simulink model "SIMULINK"  (R2024b)
settings: Solver=FixedStepDiscrete  StartTime=0.0  StopTime=inf  FixedStep=0.01  RelTol=1e-3
undefined symbols (not defined in the file or in its folder): canChannel
libraries: canlib x7, canmsglib x6
settings Model: Creator=sg128629  LastModifiedBy=sg128629

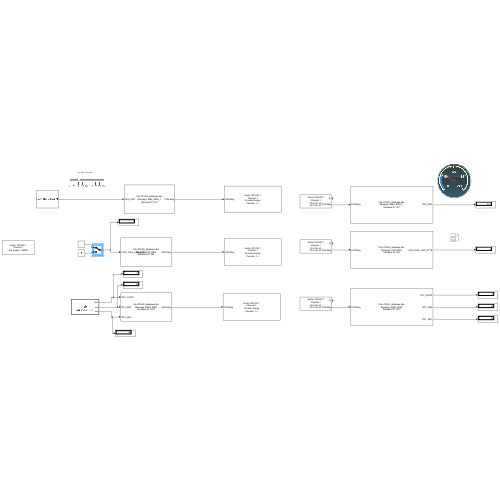
[thumbnail: Simulink's stored preview of the top-level diagram]
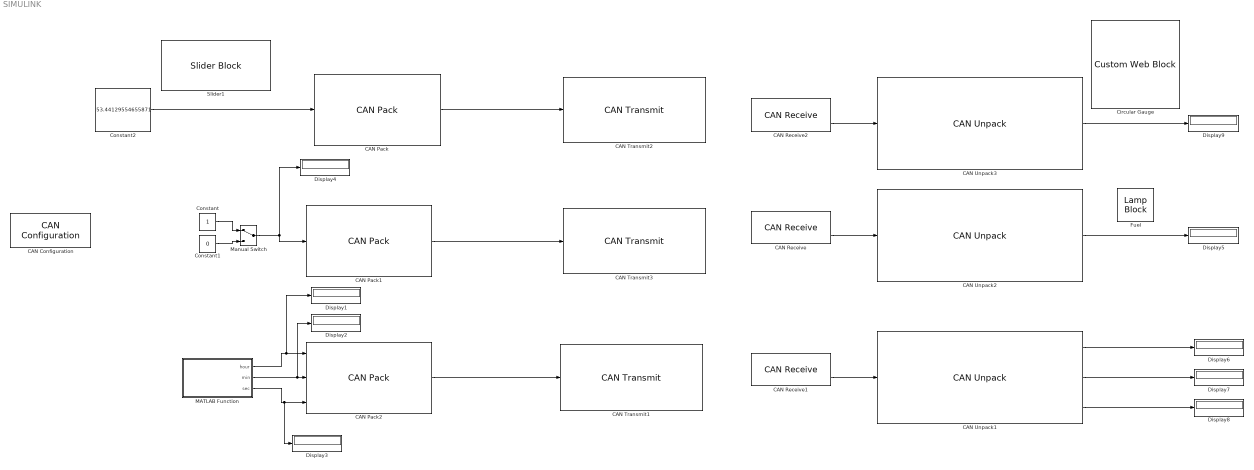
== system SIMULINK ==
  CAN Configuration : canlib/CAN Configuration  BlockHandle=154.0001  Device=Vector VN1630 1 (Channel 1)  DeviceMenu=Vector VN1630 1 (Channel 1)  ObjConstructor=canChannel('Vector', 'VN1630 1', 1)  BusSpeed=125000  EnableBitParameters=off  SJW=1  TSEG1=4  TSEG2=3  NSamples=1  AckMode=Normal
  CAN Pack : canmsglib/CAN Pack  CANdbFile=ATLAS_database.dbc  MsgList=EMS_MSG_1  MsgName=EMS_MSG_1  MsgIDType=Standard (11-bit identifier)  MsgIdentifier=257  CANIDInput=off  MsgLength=8  Remote=off  ApplyMinMax=off  BusOutput=off  SignalInfo={'VEH_SPD','0','12','LE','signed','Standard','0','0.125','0','0','511.625'}
      settings: LibrarySourceBlock=canlib/CAN Pack  DataFormat=CANdb specified signals
  CAN Pack1 : canmsglib/CAN Pack  CANdbFile=ATLAS_database.dbc  MsgList=ICM_MSG  MsgName=ICM_MSG  MsgIDType=Standard (11-bit identifier)  MsgIdentifier=544  CANIDInput=off  MsgLength=8  Remote=off  ApplyMinMax=off  BusOutput=off  SignalInfo={'LOW_FUEL_LMP_STTS','6','2','LE','unsigned','Standard','0','1','0','-Inf','Inf'}
      settings: LibrarySourceBlock=canlib/CAN Pack  DataFormat=CANdb specified signals
  CAN Pack2 : canmsglib/CAN Pack  CANdbFile=ATLAS_database.dbc  MsgList=MMU_MSG  MsgName=MMU_MSG  MsgIDType=Standard (11-bit identifier)  MsgIdentifier=1072  CANIDInput=off  MsgLength=8  Remote=off  ApplyMinMax=off  BusOutput=off  SignalInfo={'RTC_HOUR','16','6','LE','signed','Standard','0','1','0','-Inf','Inf';'RTC_MIN','8','8','LE','signed','Standard','0','1','0','-Inf','Inf';'RTC_SEC','0','8','LE','signed','Standard','0','1','0','-Inf','Inf'}
      settings: LibrarySourceBlock=canlib/CAN Pack  DataFormat=CANdb specified signals
  CAN Receive : canlib/CAN Receive  BlockHandle=166.0001  Device=Vector VN1630 1 (Channel 1)  DeviceMenu=Vector VN1630 1 (Channel 1)  ObjConstructor=canChannel('Vector', 'VN1630 1', 1)  EnableStandardIDsFilter=off  StdIDsCombo=Allow all  StandardIDs=0  EnableExtendedIDsFilter=off  ExtIDsCombo=Allow all  ExtendedIDs=0  SampleTime=0.01  MsgsPerTimestep=1  InternalFilterUpdateStatus=on  BusOutput=off
  CAN Receive1 : canlib/CAN Receive  BlockHandle=169.0001  Device=Vector VN1630 1 (Channel 1)  DeviceMenu=Vector VN1630 1 (Channel 1)  ObjConstructor=canChannel('Vector', 'VN1630 1', 1)  EnableStandardIDsFilter=off  StdIDsCombo=Allow all  StandardIDs=0  EnableExtendedIDsFilter=off  ExtIDsCombo=Allow all  ExtendedIDs=0  SampleTime=0.01  MsgsPerTimestep=1  InternalFilterUpdateStatus=on  BusOutput=off
  CAN Receive2 : canlib/CAN Receive  BlockHandle=172.0001  Device=Vector VN1630 1 (Channel 1)  DeviceMenu=Vector VN1630 1 (Channel 1)  ObjConstructor=canChannel('Vector', 'VN1630 1', 1)  EnableStandardIDsFilter=off  StdIDsCombo=Allow all  StandardIDs=0  EnableExtendedIDsFilter=off  ExtIDsCombo=Allow all  ExtendedIDs=0  SampleTime=0.01  MsgsPerTimestep=1  InternalFilterUpdateStatus=on  BusOutput=off
  CAN Transmit1 : canlib/CAN Transmit  BlockHandle=175.0001  Device=Vector VN1630 1 (Channel 1)  DeviceMenu=Vector VN1630 1 (Channel 1)  ObjConstructor=canChannel('Vector', 'VN1630 1', 1)  EnableEventTransmit=on  EnablePeriodicTransmit=on  MessagePeriod=1.000
  CAN Transmit2 : canlib/CAN Transmit  BlockHandle=177.0001  Device=Vector VN1630 1 (Channel 1)  DeviceMenu=Vector VN1630 1 (Channel 1)  ObjConstructor=canChannel('Vector', 'VN1630 1', 1)  EnableEventTransmit=on  EnablePeriodicTransmit=on  MessagePeriod=1.000
  CAN Transmit3 : canlib/CAN Transmit  BlockHandle=179.0001  Device=Vector VN1630 1 (Channel 1)  DeviceMenu=Vector VN1630 1 (Channel 1)  ObjConstructor=canChannel('Vector', 'VN1630 1', 1)  EnableEventTransmit=on  EnablePeriodicTransmit=on  MessagePeriod=1.000
  CAN Unpack1 : canmsglib/CAN Unpack  CANdbFile=ATLAS_database.dbc  MsgList=MMU_MSG  MsgName=MMU_MSG  MsgIDType=Standard (11-bit identifier)  MsgIdentifier=1072  MsgLength=8  SignalInfo={'RTC_HOUR','16','6','LE','signed','Standard','0','1','0','-Inf','Inf';'RTC_MIN','8','8','LE','signed','Standard','0','1','0','-Inf','Inf';'RTC_SEC','0','8','LE','signed','Standard','0','1','0','-Inf','Inf'}  IDPort=off  TimestampPort=off  ErrorPort=off  RemotePort=off  LengthPort=off  StatusPort=off  ApplyMinMax=off
      settings: LibrarySourceBlock=c2000lib/Target Communication/CAN Unpack  DataFormat=CANdb specified signals
  CAN Unpack2 : canmsglib/CAN Unpack  CANdbFile=ATLAS_database.dbc  MsgList=ICM_MSG  MsgName=ICM_MSG  MsgIDType=Standard (11-bit identifier)  MsgIdentifier=544  MsgLength=8  SignalInfo={'LOW_FUEL_LMP_STTS','6','2','LE','unsigned','Standard','0','1','0','-Inf','Inf'}  IDPort=off  TimestampPort=off  ErrorPort=off  RemotePort=off  LengthPort=off  StatusPort=off  ApplyMinMax=off
      settings: LibrarySourceBlock=c2000lib/Target Communication/CAN Unpack  DataFormat=CANdb specified signals
  CAN Unpack3 : canmsglib/CAN Unpack  CANdbFile=ATLAS_database.dbc  MsgList=EMS_MSG_1  MsgName=EMS_MSG_1  MsgIDType=Standard (11-bit identifier)  MsgIdentifier=257  MsgLength=8  SignalInfo={'VEH_SPD','0','12','LE','signed','Standard','0','0.125','0','0','511.625'}  IDPort=off  TimestampPort=off  ErrorPort=off  RemotePort=off  LengthPort=off  StatusPort=off  ApplyMinMax=off
      settings: LibrarySourceBlock=c2000lib/Target Communication/CAN Unpack  DataFormat=CANdb specified signals
  Circular Gauge : CustomWebBlock  LabelPosition=Hide  ShowInitialText=on  Configuration="{\"components\":[{\"name\":\"CircularScaleComponent\",\"settings\":{\"bounds\":{\"max\":200,\"min\":0,\"tickInterval\":\"auto\"},\"direction\":\"cw\",\"flipLimits\":0,\"innerRadius\":0.75,\"internalTickHeightScaleFactor\":1,\"labelColor\":[255,255,200],\"labelFont\":{\"font\":\"Arial\",\"fontSize\":12},\"labelRadius\":0.528,\"labelTransparency\":1,\"minorTickHeightScaleFactor\":0.2,\"needleImage\":{\"size\":[200,50],\"src\":\"data:image\\/svg+xml;base64,PD94bWwgdmVyc2lvbj0iMS4wIiBlbmNvZGluZz0idXRmLTgiPz4KPCEtLSBHZW5lcmF0b3I6IEFkb2JlIElsbHVzdHJhdG9yIDI0LjEuMiwgU1ZHIEV4cG9ydCBQbHVnLUluIC4gU1ZHIFZlcnNpb246IDYuMDAgQnVpbGQgMCkgIC0tPgo8c3ZnIHZlcnNpb249IjEuMSIgaWQ9IkxheWVyXzEiIHhtbG5zPSJodHRwOi8vd3d3LnczLm9yZy8yMDAwL3N2ZyIgeG1sbnM6eGxpbms9Imh0dHA6Ly93d3cudzMub3JnLzE5OTkveGxpbmsiIHg9IjBweCIgeT0iMHB4IgoJIHZpZXdCb3g9IjAgMCAyMDAgNTAiIHN0eWxlPSJlbmFibGUtYmFja2dyb3VuZDpuZXcgMCAwIDIwMCA1MDsiIHhtbDpzcGFjZT0icHJlc2VydmUiPgo8c3R5bGUgdHlwZT0idGV4dC9jc3MiPgoJLnN0MHtmaWxsOiNFQzIxMjc7fQo8L3N0eWxlPgo8cGF0aCBjbGFzcz0ic3QwIiBkPSJNMTYyLjgsMTMuN0MxNjksNC40LDE4MS43LDEuOSwxOTEsOC4xczExLjgsMTguOSw1LjYsMjguMnMtMTguOSwxMS44LTI4LjIsNS42bDAsMAoJQzE1OS4xLDM1LjYsMTU2LjYsMjMsMTYyLjgsMTMuN0wxNjIuOCwxMy43eiBNMTY1LjgsMTUuOGMtNS4xLDcuNi0zLjEsMTcuOSw0LjYsMjNjNy42LDUuMSwxNy45LDMuMSwyMy00LjYKCWM1LjEtNy42LDMuMS0xNy45LTQuNi0yM2wwLDBDMTgxLjIsNi4yLDE3MC45LDguMiwxNjUuOCwxNS44eiIvPgo8cGF0aCBjbGFzcz0ic3QwIiBkPSJNMC40LDI1Ljl2LTMuM2wxNTktMi41Yy0wLjcsMi42LTAuNyw1LjIsMCw3LjhMMC40LDI1Ljl6Ii8+CjxjaXJjbGUgY2xhc3M9InN0MCIgY3g9IjE3OS42IiBjeT0iMjQiIHI9IjAuNyIvPgo8L3N2Zz4K\"},\"needleOffset\":[0.18464878250906522,0],\"needleOrientation\":-45,\"needleRotation\":180,\"needleSize\":{\"height\":0.11741692305346914,\"width\":0.46108337545091255},\"outerRadius\":0.9,\"position\":[0.029134114583333332,0.03955078125,0.89990234375,0.89990234375],\"referencePoint\":\"auto\",\"scaleAngle\":270,\"scaleAngleOffset\":135,\"scaleColors\":[],\"scaleColorsSize\":0.2,\"scaleDirection\":\"CW\",\"scalePosition\":[0,0,1,1],\"showLabels\":1,\"showMinorTicks\":1,\"showSpanLine\":1,\"showTicks\":1,\"tickColor\":[252,252,197],\"tickTransparency\":1,\"valueBarColor\":[0,114,189],\"valueBarPosition\":[0,0,1,1],\"valueBarSize\":0.2,\"valueBarTransparency\":1}},{\"name\":\"BackgroundImageComponent\",\"settings\":{\"image\":{\"size\":[500,500],\"src\":\"data:image\\/svg+xml;base64,PD94bWwgdmVyc2lvbj0iMS4wIiBlbmNvZGluZz0iVVRGLTgiIHN0YW5kYWxvbmU9Im5vIj8+CjxzdmcKICAgeG1sbnM6ZGM9Imh0dHA6Ly9wdXJsLm9yZy9kYy9lbGVtZW50cy8xLjEvIgogICB4bWxuczpjYz0iaHR0cDovL2NyZWF0aXZlY29tbW9ucy5vcmcvbnMjIgogICB4bWxuczpyZGY9Imh0dHA6Ly93d3cudzMub3JnLzE5OTkvMDIvMjItcmRmLXN5bnRheC1ucyMiCiAgIHhtbG5zOnN2Zz0iaHR0cDovL3d3dy53My5vcmcvMjAwMC9zdmciCiAgIHhtbG5zPSJodHRwOi8vd3d3LnczLm9yZy8yMDAwL3N2ZyIKICAgeG1sbnM6 ...(+9964 chars)\"},\"position\":[0,0,1,1],\"scaleMode\":\"0\"}},{\"name\":\"ForegroundImageComponent\",\"settings\":{\"image\":{\"size\":[0,0],\"src\":\"default\",\"srcOrientation\":[]},\"isForeground\":1,\"position\":[0,0,1,1],\"scaleMode\":\"0\"}}],\"settings\":{\"BindingType\":\"signal\",\"aspectRatio\":1.032258064516129,\"backgroundColor\":[0,0,0,\"1\"],\"backgroundOffset\":1,\"backgroundOpacity\":1,\"direction\":\"cw\",\"fixedAspectRatio\":\"on\",\"flipLimits\":0,\"orientation\":\"horizontal\",\"showBackgroundColor\":false,\"value\":0,\"version\":\"R2023a\"},\"type\":\"CircularGauge\"}"
  Constant : Constant
  Constant1 : Constant  Value=0
  Constant2 : Constant  Value=53.44129554655871  SampleTime=1
  Display{1..9} (9 alike) : Display
  Fuel : LampBlock  LabelPosition=Hide  Icon=Fuel
  MATLAB Function : MATLAB Function  TreatAsAtomicUnit=on
  Manual Switch : ManualSwitch
  Slider1 : SliderBlock  ScaleMax=200
  wires:
  CAN Pack2/1 -> CAN Transmit1/1
  MATLAB Function/3(sec) -> Display3/1, CAN Pack2/3
  MATLAB Function/1(hour) -> Display1/1, CAN Pack2/1
  MATLAB Function/2(min) -> Display2/1, CAN Pack2/2
  CAN Pack/1 -> CAN Transmit2/1
  CAN Pack1/1 -> CAN Transmit3/1
  Constant/1 -> Manual Switch/1
  Manual Switch/1 -> Display4/1, CAN Pack1/1
  Constant1/1 -> Manual Switch/2
  CAN Unpack2/1 -> Display5/1
  CAN Receive/2 -> CAN Unpack2/1
  CAN Receive1/2 -> CAN Unpack1/1
  CAN Unpack1/1 -> Display6/1
  CAN Unpack1/2 -> Display7/1
  CAN Unpack1/3 -> Display8/1
  CAN Receive2/2 -> CAN Unpack3/1
  CAN Unpack3/1 -> Display9/1
  Constant2/1 -> CAN Pack/1

== matlab function SIMULINK/MATLAB Function ==
  data: hour output; min output; sec output
function [hour, min, sec] = get_system_time()
    % Read current system time
    c = clock;  % Returns [year month day hour min sec]

    hour = uint8(c(4));       % Extract hour (0-23)
    min  = uint8(c(5));       % Extract minute (0-59)
    sec  = uint8(floor(c(6))); % Extract seconds (floor to integer 0-59)
end
